simulink model "sf_edge_triggered_output_event"  (R2025b)
settings: Solver=FixedStepDiscrete  StartTime=0.0  StopTime=4  FixedStep=0.1  MaxStep=.1  RelTol=1e-3  EnableMultiTasking=on
settings Model: Creator=The MathWorks, Inc.  LastModifiedBy=The MathWorks, Inc.
settings SolverCC: AlgebraicLoopSolver=TrustRegion
settings DataIOCC: LimitDataPoints=on  SaveFormat=Array  ReturnWorkspaceOutputs=off
settings OptimizationCC: ReuseModelBlockBuffer=off  ExpressionDepthLimit=2147483647.0  InitFltsAndDblsToZero=on  EfficientMapNaN2IntZero=off  LifeSpan=inf
settings DebuggingCC: SaveWithParameterizedLinksMsg=none  UnderspecifiedInitializationDetection=Classic  MergeDetectMultiDrivingBlocksExec=none  SolverPrmCheckMsg=warning  FcnCallInpInsideContextMsg=warning  UnconnectedInputMsg=warning  UnconnectedOutputMsg=warning  UnconnectedLineMsg=warning  StateNameClashWarn=warning  SFUnexpectedBacktrackingDiag=warning  SFNoUnconditionalDefaultTransitionDiag=warning  SFExecutionAtInitializationDiag=none  ArithmeticOperatorsInVariantConditions=warning
settings HardwareCC: ProdBitPerPointer=32.0  ProdBitPerSizeT=32.0  ProdBitPerPtrDiffT=32.0  ProdLargestAtomicFloat=None  ProdIntDivRoundTo=Undefined  ProdEndianess=Unspecified  ProdWordSize=32.0  ProdHWDeviceType=32-bit Generic
settings ModelReferenceCC: EnableRefExpFcnMdlSchedulingChecks=on  PropagateSignalLabelsOutOfModel=off
settings SFSimCC: SimUseLocalCustomCode=off  SimParseCustomCode=off  CustomCodeUndefinedFunction=UseInterfaceOnly
settings RTWCC: RTWUseLocalCustomCode=off  GPUComputeCapability=3.5
settings CodeAppCC: StateflowObjectComments=on
settings GRTTargetCC: TargetFcnLib=ansi_tfl_tmw.mat  TargetLangStandard=C89/C90 (ANSI)  CombineOutputUpdateFcns=off  GRTInterface=on
settings ConfigComp: CovMetricSettings=dw  CovSaveCumulativeToWorkspaceVar=on  CovSaveSingleToWorkspaceVar=on  CovExternalEMLEnable=off

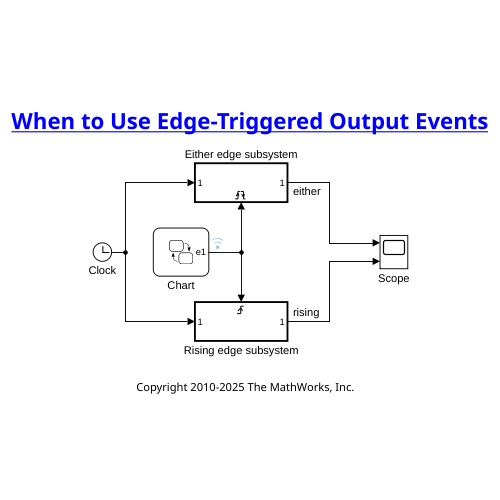
[thumbnail: Simulink's stored preview of the top-level diagram]
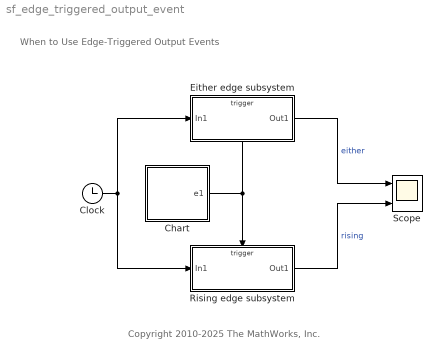
== system sf_edge_triggered_output_event ==
  note: Copyright 2010-2025 The MathWorks, Inc.
  note: When to Use Edge-Triggered Output Events
  Chart : Stateflow chart  TreatAsAtomicUnit=on
  Clock : Clock
  Either edge subsystem : Subsystem  TreatAsAtomicUnit=on
  Rising edge subsystem : Subsystem  TreatAsAtomicUnit=on
  Scope : Scope  NumInputPorts=2
      settings: TimeSpan=4  ActiveDisplayYMinimum=0  ActiveDisplayYMaximum=4
  wires:
  Chart/1(e1) -> Rising edge subsystem/Trigger, Either edge subsystem/Trigger
  Clock/1 -> Rising edge subsystem/1(In1), Either edge subsystem/1(In1)
  Rising edge subsystem/1(Out1) -> Scope/2  "rising"
  Either edge subsystem/1(Out1) -> Scope/1  "either"

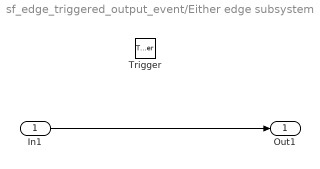
== system sf_edge_triggered_output_event/Either edge subsystem ==
  In1 : Inport
  Trigger : TriggerPort  TriggerType=either  VariantControl=Variant
  Out1 : Outport  VectorParamsAs1DForOutWhenUnconnected=off
  wires:
  In1/1 -> Out1/1

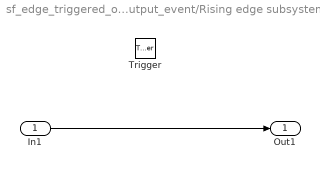
== system sf_edge_triggered_output_event/Rising edge subsystem ==
  In1 : Inport
  Trigger : TriggerPort  VariantControl=Variant
  Out1 : Outport  VectorParamsAs1DForOutWhenUnconnected=off
  wires:
  In1/1 -> Out1/1

== stateflow chart sf_edge_triggered_output_event/Chart ==
  state A
    du: a=1;
  state B
    en: send(e1);
    du: a=0;
  (default) -> A
  A -> B : [a==1]
  B -> A : [a==0]
  data: a local double
  events: e1 output EITHER_EDGE_EVENT
